simulink model "plantaCPC_2025_PLC"  (R2025b)
settings: Solver=ode45  StartTime=0.0  StopTime=300  MaxStep=0.01  RelTol=1e-5  EnableMultiTasking=on
values from neighbouring files (symbols this model uses):
  A = 0.159    [Fuzzy_no_anfis_sim.m]    (also in build_FLC_L4_anfis.m = zeros(size(Xtr,1), nOut); build_FLC_lower_single.m; build_FLC_upper_single.m; fuzzym.m)
  a1 = 6.1360e-04    (= 0.0006136)    [Fuzzy_no_anfis_sim.m]    (also in build_FLC_lower_single.m; fuzzym.m)
  a2 = 5.4678e-04    (= 0.00054678)    [Fuzzy_no_anfis_sim.m]    (also in build_FLC_lower_single.m; fuzzym.m)
  a3 = 3.5752e-04    (= 0.00035752)    [Fuzzy_no_anfis_sim.m]    (also in build_FLC_lower_single.m; fuzzym.m)
  a4 = 4.1820e-04    (= 0.0004182)    [Fuzzy_no_anfis_sim.m]    (also in build_FLC_L4_anfis.m; build_FLC_L4_single.m; build_FLC_lower_single.m; fuzzym.m)
  dumax = 1    [Fuzzy_no_anfis_sim.m]
  gamma1 = 0.455    [Fuzzy_no_anfis_sim.m]    (also in build_FLC_L4_anfis.m; build_FLC_L4_single.m; build_FLC_lower_single.m; fuzzym.m)
  gamma2 = 0.4195    [Fuzzy_no_anfis_sim.m]    (also in build_FLC_lower_single.m; fuzzym.m)
  k1 = q_max    (= 0.0017)    [Fuzzy_no_anfis_sim.m]    (also in build_FLC_L4_anfis.m; build_FLC_L4_single.m; fuzzym.m)
  k2 = q_max    (= 0.0017)    [Fuzzy_no_anfis_sim.m]    (also in fuzzym.m)
  Ts = 0.1    [Fuzzy_no_anfis_sim.m]    (also in build_FLC_L4_single.m; build_FLC_lower_single.m; build_FLC_upper_single.m; deadbeat_flc_pump2.m = 1)
undefined symbols (not defined in the file or in its folder): dspblkCoreblockFVToolHelper, gcbh
libraries: simulink x30, fuzblock x4
settings Model: PacingRate=3  Creator=Administrator  LastModifiedBy=wepi
settings DataIOCC: LimitDataPoints=on  SaveFormat=Array  ReturnWorkspaceOutputs=off
settings OptimizationCC: LifeSpan=inf
settings DebuggingCC: UnderspecifiedInitializationDetection=Classic  MergeDetectMultiDrivingBlocksExec=none  SolverPrmCheckMsg=warning  UnconnectedInputMsg=warning  UnconnectedOutputMsg=warning  UnconnectedLineMsg=warning  StateNameClashWarn=warning  SFUnexpectedBacktrackingDiag=warning  SFNoUnconditionalDefaultTransitionDiag=warning  SFExecutionAtInitializationDiag=none  ArithmeticOperatorsInVariantConditions=warning
settings HardwareCC: ProdBitPerPointer=32.0  ProdBitPerSizeT=32.0  ProdBitPerPtrDiffT=32.0  ProdLargestAtomicFloat=None  ProdIntDivRoundTo=Undefined  ProdEndianess=Unspecified  ProdWordSize=32.0  ProdHWDeviceType=32-bit Generic
settings ModelReferenceCC: PropagateSignalLabelsOutOfModel=off
settings SFSimCC: SimUseLocalCustomCode=off  CustomCodeUndefinedFunction=UseInterfaceOnly
settings RTWCC: RTWUseLocalCustomCode=off  GPUComputeCapability=3.5
settings CodeAppCC: StateflowObjectComments=on
settings GRTTargetCC: TargetLangStandard=C89/C90 (ANSI)
settings ConfigComp: CovMetricSettings=dw  CovSaveCumulativeToWorkspaceVar=on  CovSaveSingleToWorkspaceVar=on  CovExternalEMLEnable=off

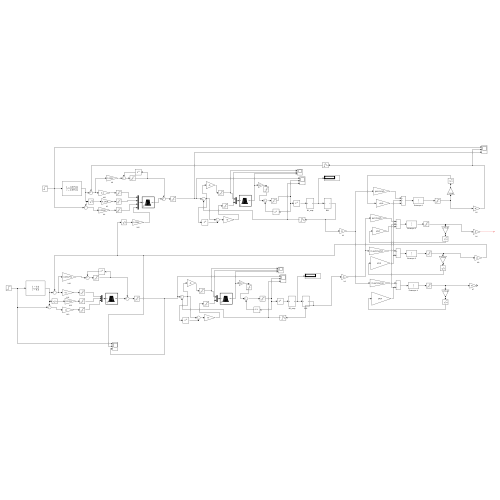
[thumbnail: Simulink's stored preview of the top-level diagram]
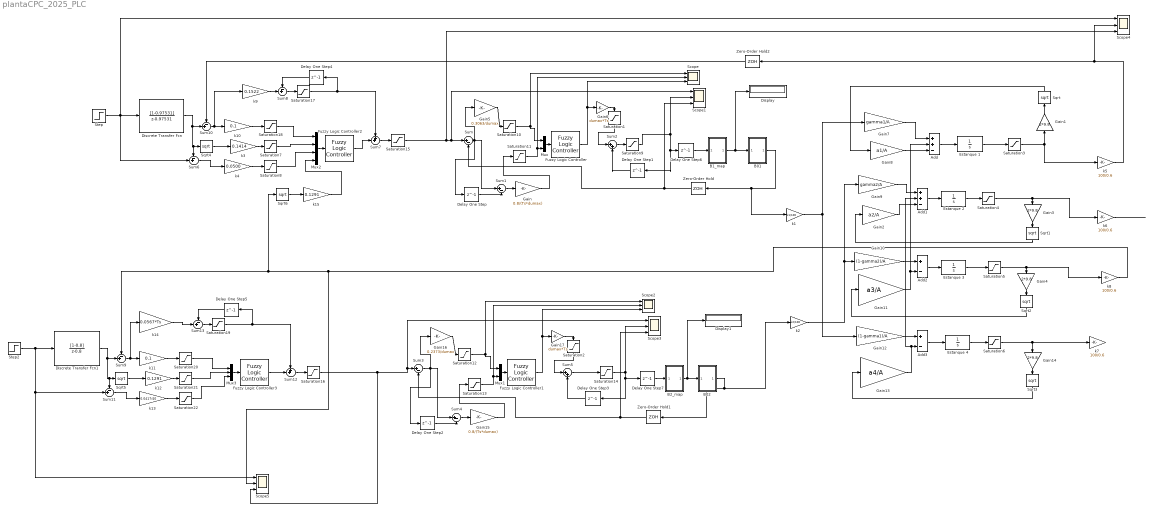
== system plantaCPC_2025_PLC ==
  Add : Sum  Inputs=++-
  Add1 : Sum  Inputs=++-
  Add2 : Sum  Inputs=+-
  Add3 : Sum  Inputs=+-
  B01 : Subsystem
  B02 : Subsystem
  B1_map : Subsystem
  B2_map : Subsystem
  Delay One Step{,2,6..7} (4 alike) : Delay  DelayLength=1  SampleTime=0.1
  Delay One Step1 : Delay  DelayLength=1  InitialCondition=0  SampleTime=0.1
  Delay One Step3 : Delay  DelayLength=1  InitialCondition=40  SampleTime=0.1
  Delay One Step4 : Delay  DelayLength=1  InitialCondition=0  SampleTime=0.1
  Delay One Step5 : Delay  DelayLength=1  InitialCondition=0  SampleTime=0.1
  Discrete Transfer Fcn : DiscreteTransferFcn  LoadFcn=dspblkCoreblockFVToolHelper(gcbh,'load');  Numerator=[1-0.97531]  Denominator=[1 -0.97531]
      settings: CopyFcn=dspblkCoreblockFVToolHelper(gcbh,'copy');  DeleteFcn=dspblkCoreblockFVToolHelper(gcbh,'close');  ModelCloseFcn=dspblkCoreblockFVToolHelper(gcbh,'close');  PreSaveFcn=dspblkCoreblockFVToolHelper(gcbh,'presave');  PostSaveFcn=dspblkCoreblockFVToolHelper(gcbh,'postsave');  CloseFcn=dspblkCoreblockFVToolHelper(gcbh,'close');
  Discrete Transfer Fcn1 : DiscreteTransferFcn  LoadFcn=dspblkCoreblockFVToolHelper(gcbh,'load');  Numerator=[1-0.8]  Denominator=[1 -0.8]
      settings: CopyFcn=dspblkCoreblockFVToolHelper(gcbh,'copy');  DeleteFcn=dspblkCoreblockFVToolHelper(gcbh,'close');  ModelCloseFcn=dspblkCoreblockFVToolHelper(gcbh,'close');  PreSaveFcn=dspblkCoreblockFVToolHelper(gcbh,'presave');  PostSaveFcn=dspblkCoreblockFVToolHelper(gcbh,'postsave');  CloseFcn=dspblkCoreblockFVToolHelper(gcbh,'close');
  Display : Display
  Display1 : Display
  Estanque 1 : TransferFcn  Denominator=[1 0]
  "Estanque 2 " : TransferFcn  Denominator=[1 0]
  Estanque 3 : TransferFcn  Denominator=[1 0]
  Estanque 4 : TransferFcn  Denominator=[1 0]
  Fuzzy Logic Controller : fuzblock/Fuzzy Logic  Controller  FIS=FLC_F1  OutputSampleNumber=101  DataType=double  UseLookupTable=off  NumBreakpoints=10  FuzzifiedInputs=off  RuleFiringStrengths=off  RuleOutputs=off  AggregatedOutputs=off  SimulateUsing=Interpreted execution  OutOfRangeInputValueMessage=warning  NoRuleFiredMessage=warning  EmptyOutputFuzzySetMessage=warning
  Fuzzy Logic Controller1 : fuzblock/Fuzzy Logic  Controller  FIS=FLC_F2  OutputSampleNumber=101  DataType=double  UseLookupTable=off  NumBreakpoints=10  FuzzifiedInputs=off  RuleFiringStrengths=off  RuleOutputs=off  AggregatedOutputs=off  SimulateUsing=Interpreted execution  OutOfRangeInputValueMessage=warning  NoRuleFiredMessage=warning  EmptyOutputFuzzySetMessage=warning
  Fuzzy Logic Controller2 : fuzblock/Fuzzy Logic  Controller  FIS=FLC_L1  OutputSampleNumber=101  DataType=double  UseLookupTable=off  NumBreakpoints=10  FuzzifiedInputs=off  RuleFiringStrengths=off  RuleOutputs=off  AggregatedOutputs=off  SimulateUsing=Interpreted execution  OutOfRangeInputValueMessage=warning  NoRuleFiredMessage=warning  EmptyOutputFuzzySetMessage=warning
  Fuzzy Logic Controller3 : fuzblock/Fuzzy Logic  Controller  FIS=FLC_L3  OutputSampleNumber=101  DataType=double  UseLookupTable=off  NumBreakpoints=10  FuzzifiedInputs=off  RuleFiringStrengths=off  RuleOutputs=off  AggregatedOutputs=off  SimulateUsing=Interpreted execution  OutOfRangeInputValueMessage=warning  NoRuleFiredMessage=warning  EmptyOutputFuzzySetMessage=warning
  Gain : Gain  Gain=0.8/(Ts*dumax)
  Gain{1,3..4,14} (4 alike) : Gain  Gain=2*9.8
  Gain10 : Gain  Gain=(1-gamma2)/A
  Gain11 : Gain  Gain=a3/A
  Gain12 : Gain  Gain=(1-gamma1)/A
  Gain13 : Gain  Gain=a4/A
  Gain15 : Gain  Gain=0.8/(Ts*dumax)
  Gain16 : Gain  Gain=0.2373/dumax
  Gain17 : Gain  Gain=dumax*Ts
  Gain2 : Gain  Gain=a2/A
  Gain5 : Gain  Gain=0.3063/dumax
  Gain6 : Gain  Gain=dumax*Ts
  Gain7 : Gain  Gain=gamma1/A
  Gain8 : Gain  Gain=a1/A
  Gain9 : Gain  Gain=gamma2/A
  Mux : Mux  Inputs=2
  Mux1 : Mux  Inputs=2
  Mux2 : Mux
  Mux3 : Mux  Inputs=3
  Saturation1 : Saturate  UpperLimit=dumax*Ts  LowerLimit=-dumax*Ts
  Saturation{8,10..13,18,20,22} (8 alike) : Saturate  UpperLimit=1  LowerLimit=-1
  Saturation{9,14..16} (4 alike) : Saturate  UpperLimit=100  LowerLimit=0
  Saturation17 : Saturate  UpperLimit=30  LowerLimit=-30
  Saturation19 : Saturate  UpperLimit=30  LowerLimit=-30
  Saturation2 : Saturate  UpperLimit=dumax*Ts  LowerLimit=-dumax*Ts
  Saturation21 : Saturate  UpperLimit=1  LowerLimit=0
  Saturation{3..6} (4 alike) : Saturate  UpperLimit=0.8  LowerLimit=0
  Saturation7 : Saturate  UpperLimit=1  LowerLimit=0
  Scope{,1..5} (6 alike) : Scope  NumInputPorts=3
      Scope settings: ActiveDisplayYMinimum=103.80137956396959  ActiveDisplayYMaximum=139.96234120398589
      Scope1 settings: ActiveDisplayYMinimum=-68.909700061778238  ActiveDisplayYMaximum=113.12239490018993
      Scope2 settings: ActiveDisplayYMinimum=103.80137956396959  ActiveDisplayYMaximum=139.96234120398589  DataLoggingVariableName=ScopeData2
      Scope3 settings: ActiveDisplayYMinimum=-52.0727443173749  ActiveDisplayYMaximum=103.1546988563742  DataLoggingVariableName=ScopeData3
      Scope4 settings: ActiveDisplayYMinimum=-77.521735134950461  ActiveDisplayYMaximum=137.02283230652165  DataLoggingVariableName=ScopeData4
      Scope5 settings: ActiveDisplayYMinimum=-10.950989781729737  ActiveDisplayYMaximum=98.55890803556764  DataLoggingVariableName=ScopeData5
  Sqrt{,1..6} (7 alike) : Sqrt
  Step : Step  Time=200  Before=10  After=20  SampleTime=0
  Step2 : Step  Time=90  Before=10  After=20  SampleTime=0
  Sum{,1,3..4} (4 alike) : Sum  Inputs=|+-
  Sum{6,8..11,13} (6 alike) : Sum  Inputs=-+|
  Sum12 : Sum  Inputs=++|
  Sum2 : Sum  Inputs=|++
  Sum5 : Sum  Inputs=|++
  Sum7 : Sum  Inputs=++|
  Zero-Order Hold : ZeroOrderHold  SampleTime=Ts
  Zero-Order Hold1 : ZeroOrderHold  SampleTime=Ts
  Zero-Order Hold2 : ZeroOrderHold  SampleTime=Ts
  k1 : Gain  Gain=k1/100
  k10 : Gain  Gain=0.1
  k11 : Gain  Gain=0.1
  k12 : Gain  Gain=0.1291
  k13 : Gain  Gain=0.0417/40
  k14 : Gain  Gain=0.0567*Ts
  k15 : Gain  Gain=0.1291
  k2 : Gain  Gain=k2/100
  k3 : Gain  Gain=0.1414
  k4 : Gain  Gain=0.0500
  k{5..8} (4 alike) : Gain  Gain=100/0.6
  k9 : Gain  Gain=0.1522
  wires:
  Saturation3/1 -> k5/1, Gain1/1
  Saturation4/1 -> k6/1, Gain3/1
  Saturation5/1 -> k8/1, Gain4/1
  Estanque 1/1 -> Saturation3/1
  "Estanque 2 "/1 -> Saturation4/1
  Estanque 4/1 -> Saturation6/1
  Fuzzy Logic Controller/1 -> Gain6/1, Scope/3
  Gain7/1 -> Add/1
  k1/1 -> Gain12/1, Gain7/1
  Gain8/1 -> Add/3
  Add/1 -> Estanque 1/1
  Add1/1 -> "Estanque 2 "/1
  Add2/1 -> Estanque 3/1
  Add3/1 -> Estanque 4/1
  Gain9/1 -> Add1/1
  k2/1 -> Gain9/1, Gain10/1
  Gain2/1 -> Add1/3
  Gain10/1 -> Add2/1
  Gain11/1 -> Add/2, Add2/2
  Gain12/1 -> Add3/1
  Gain13/1 -> Add1/2, Add3/2
  Estanque 3/1 -> Saturation5/1
  Gain1/1 -> Sqrt/1
  Sqrt/1 -> Gain8/1
  Gain3/1 -> Sqrt1/1
  Sqrt1/1 -> Gain2/1
  Gain4/1 -> Sqrt2/1
  Gain14/1 -> Sqrt3/1
  Saturation6/1 -> Gain14/1, k7/1
  Sqrt3/1 -> Gain13/1
  Sqrt2/1 -> Gain11/1
  Sum2/1 -> Saturation9/1
  k6/1 -> ?
  Sum/1 -> Delay One Step/1, Gain5/1, Sum1/1
  Mux/1 -> Fuzzy Logic Controller/1
  Delay One Step/1 -> Sum1/2
  Saturation11/1 -> Scope/2, Mux/2
  Saturation10/1 -> Scope/1, Mux/1
  Saturation9/1 -> Delay One Step1/1, Delay One Step6/1, Scope1/2
  B01/1(Out1) -> k1/1, Zero-Order Hold/1
  Gain6/1 -> Saturation1/1
  Saturation1/1 -> Sum2/1
  Delay One Step1/1 -> Sum2/2
  Gain5/1 -> Saturation10/1
  Sum1/1 -> Gain/1
  Gain/1 -> Saturation11/1
  B1_map/1(Out1) -> Display/1, B01/1(In1)
  Zero-Order Hold/1 -> Sum/2, Scope1/3
  Mux1/1 -> Fuzzy Logic Controller1/1
  Sum5/1 -> Saturation14/1
  Delay One Step3/1 -> Sum5/2
  Sum4/1 -> Gain15/1
  B2_map/1(Out1) -> Display1/1, B02/1(In1)
  Gain16/1 -> Saturation12/1
  B02/1(Out1) -> Zero-Order Hold1/1, k2/1
  Fuzzy Logic Controller1/1 -> Gain17/1, Scope2/3
  Zero-Order Hold1/1 -> Sum3/2, Scope3/3
  Sum3/1 -> Delay One Step2/1, Gain16/1, Sum4/1
  Saturation13/1 -> Scope2/2, Mux1/2
  Delay One Step2/1 -> Sum4/2
  Gain15/1 -> Saturation13/1
  Saturation16/1 -> Scope5/3, Scope3/1, Sum3/1
  Gain17/1 -> Saturation2/1
  Saturation2/1 -> Sum5/1
  Saturation12/1 -> Scope2/1, Mux1/1
  Saturation14/1 -> Delay One Step7/1, Delay One Step3/1, Scope3/2
  Mux2/1 -> Fuzzy Logic Controller2/1
  Fuzzy Logic Controller2/1 -> Sum7/2
  Saturation15/1 -> Scope4/3, Scope1/1, Sum/1
  Delay One Step6/1 -> B1_map/1(In1)
  Step/1 -> Sum6/2, Scope4/1, Discrete Transfer Fcn/1
  Discrete Transfer Fcn/1 -> Sum6/1, Sqrt4/1, Sum10/2
  Sum10/1 -> k9/1, k10/1
  k10/1 -> Saturation18/1
  Saturation18/1 -> Mux2/1
  Zero-Order Hold2/1 -> Sum10/1
  Sum7/1 -> Saturation15/1
  k3/1 -> Saturation7/1
  Saturation7/1 -> Mux2/2
  Sum6/1 -> k4/1
  k4/1 -> Saturation8/1
  Saturation8/1 -> Mux2/3
  k9/1 -> Sum8/2
  Sum8/1 -> Saturation17/1
  Saturation17/1 -> Delay One Step4/1, Sum7/1
  Delay One Step4/1 -> Sum8/1
  Sqrt4/1 -> k3/1
  Sum12/1 -> Saturation16/1
  k13/1 -> Saturation22/1
  Mux3/1 -> Fuzzy Logic Controller3/1
  k12/1 -> Saturation21/1
  Fuzzy Logic Controller3/1 -> Sum12/2
  Saturation21/1 -> Mux3/2
  Sum13/1 -> Saturation19/1
  Step2/1 -> Scope5/1, Sum11/2, Discrete Transfer Fcn1/1
  Saturation22/1 -> Mux3/3
  k14/1 -> Sum13/2
  k11/1 -> Saturation20/1
  Discrete Transfer Fcn1/1 -> Sum11/1, Sqrt5/1, Sum9/2
  Sum9/1 -> k14/1, k11/1
  Sqrt5/1 -> k12/1
  Saturation19/1 -> Delay One Step5/1, Sum12/1
  Saturation20/1 -> Mux3/1
  Delay One Step5/1 -> Sum13/1
  Sum11/1 -> k13/1
  k8/1 -> Scope5/2, Sqrt6/1, Sum9/1
  Delay One Step7/1 -> B2_map/1(In1)
  Sqrt6/1 -> k15/1
  k15/1 -> Mux2/4
  k5/1 -> Scope4/2, Zero-Order Hold2/1

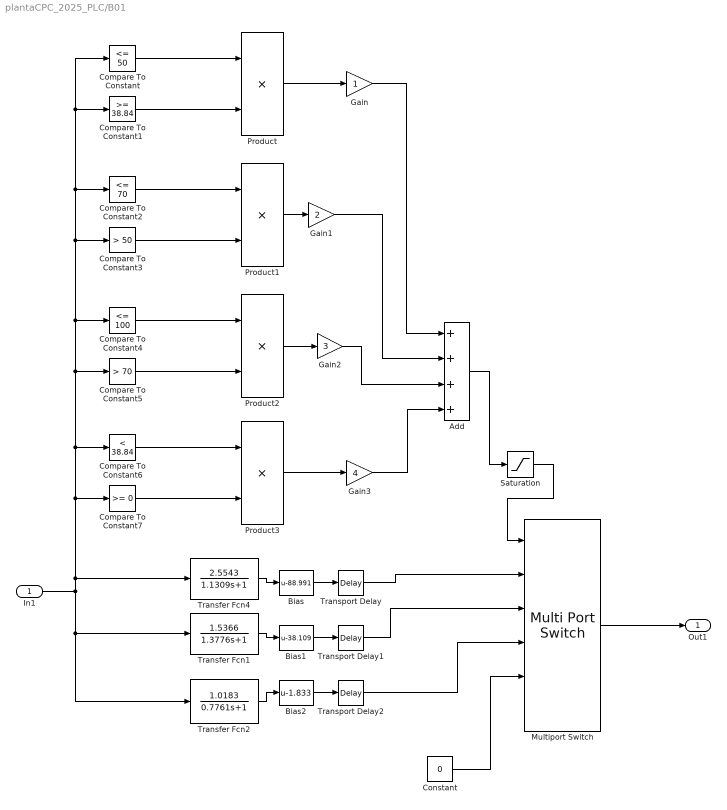
== system plantaCPC_2025_PLC/B01 ==
  In1 : Inport
  Add : Sum  Inputs=++++
  Bias : Bias  Bias=-88.991  SaturateOnIntegerOverflow=off
  Bias1 : Bias  Bias=-38.109  SaturateOnIntegerOverflow=off
  Bias2 : Bias  Bias=-1.833  SaturateOnIntegerOverflow=off
  Compare To Constant : simulink/Logic and Bit Operations/Compare To Constant  relop=<=  const=50  OutDataTypeStr=boolean
  Compare To Constant1 : simulink/Logic and Bit Operations/Compare To Constant  relop=>=  const=38.84  OutDataTypeStr=boolean
  Compare To Constant2 : simulink/Logic and Bit Operations/Compare To Constant  relop=<=  const=70  OutDataTypeStr=boolean
  Compare To Constant3 : simulink/Logic and Bit Operations/Compare To Constant  relop=>  const=50  OutDataTypeStr=boolean
  Compare To Constant4 : simulink/Logic and Bit Operations/Compare To Constant  relop=<=  const=100  OutDataTypeStr=boolean
  Compare To Constant5 : simulink/Logic and Bit Operations/Compare To Constant  relop=>  const=70  OutDataTypeStr=boolean
  Compare To Constant6 : simulink/Logic and Bit Operations/Compare To Constant  relop=<  const=38.84  OutDataTypeStr=boolean
  Compare To Constant7 : simulink/Logic and Bit Operations/Compare To Constant  relop=>=  const=0  OutDataTypeStr=boolean
  Constant : Constant  Value=0
  Gain : Gain
  Gain1 : Gain  Gain=2
  Gain2 : Gain  Gain=3
  Gain3 : Gain  Gain=4
  Multiport Switch : MultiPortSwitch  Inputs=5  SaturateOnIntegerOverflow=off  InputSameDT=off
  Product{,1..3} (4 alike) : Product
  Saturation : Saturate  UpperLimit=5  LowerLimit=1
  Transfer Fcn1 : TransferFcn  Numerator=[1.5366]  Denominator=[1.3776 1]
  Transfer Fcn2 : TransferFcn  Numerator=[1.0183]  Denominator=[0.7761 1]
  Transfer Fcn4 : TransferFcn  Numerator=[2.5543]  Denominator=[1.1309 1]
  Transport Delay : TransportDelay  DelayTime=0.6
  Transport Delay1 : TransportDelay  DelayTime=0.5
  Transport Delay2 : TransportDelay  DelayTime=0.5
  Out1 : Outport
  wires:
  Multiport Switch/1 -> Out1/1
  Product/1 -> Gain/1
  Gain/1 -> Add/1
  Product1/1 -> Gain1/1
  Gain1/1 -> Add/2
  Gain2/1 -> Add/3
  Product2/1 -> Gain2/1
  Add/1 -> Saturation/1
  Compare To Constant/1 -> Product/1
  Transfer Fcn4/1 -> Bias/1
  Transfer Fcn1/1 -> Bias1/1
  Transfer Fcn2/1 -> Bias2/1
  Compare To Constant1/1 -> Product/2
  Compare To Constant2/1 -> Product1/1
  Compare To Constant3/1 -> Product1/2
  Compare To Constant4/1 -> Product2/1
  Compare To Constant5/1 -> Product2/2
  Transport Delay1/1 -> Multiport Switch/3
  Transport Delay2/1 -> Multiport Switch/4
  Bias/1 -> Transport Delay/1
  Bias1/1 -> Transport Delay1/1
  Bias2/1 -> Transport Delay2/1
  Product3/1 -> Gain3/1
  Compare To Constant6/1 -> Product3/1
  Compare To Constant7/1 -> Product3/2
  In1/1 -> Compare To Constant7/1, Compare To Constant6/1, Compare To Constant4/1, Compare To Constant2/1, Compare To Constant1/1, Compare To Constant/1, Compare To Constant3/1, Compare To Constant5/1, Transfer Fcn4/1, Transfer Fcn2/1, Transfer Fcn1/1
  Gain3/1 -> Add/4
  Constant/1 -> Multiport Switch/5
  Transport Delay/1 -> Multiport Switch/2
  Saturation/1 -> Multiport Switch/1

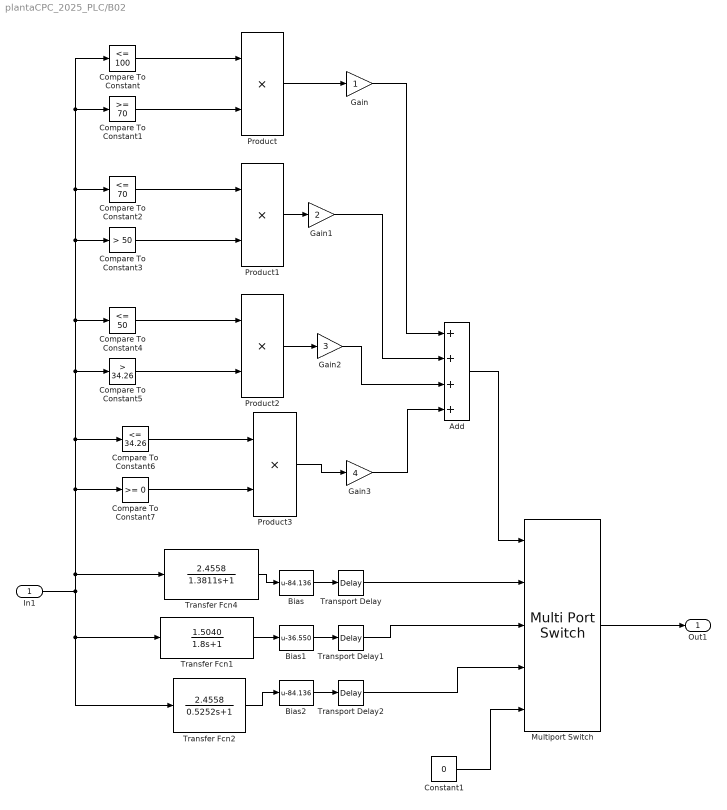
== system plantaCPC_2025_PLC/B02 ==
  In1 : Inport
  Add : Sum  Inputs=++++
  Bias : Bias  Bias=-84.136  SaturateOnIntegerOverflow=off
  Bias1 : Bias  Bias=-36.550  SaturateOnIntegerOverflow=off
  Bias2 : Bias  Bias=-84.136  SaturateOnIntegerOverflow=off
  Compare To Constant : simulink/Logic and Bit Operations/Compare To Constant  relop=<=  const=100  OutDataTypeStr=boolean
  Compare To Constant1 : simulink/Logic and Bit Operations/Compare To Constant  relop=>=  const=70  OutDataTypeStr=boolean
  Compare To Constant2 : simulink/Logic and Bit Operations/Compare To Constant  relop=<=  const=70  OutDataTypeStr=boolean
  Compare To Constant3 : simulink/Logic and Bit Operations/Compare To Constant  relop=>  const=50  OutDataTypeStr=boolean
  Compare To Constant4 : simulink/Logic and Bit Operations/Compare To Constant  relop=<=  const=50  OutDataTypeStr=boolean
  Compare To Constant5 : simulink/Logic and Bit Operations/Compare To Constant  relop=>  const=34.26  OutDataTypeStr=boolean
  Compare To Constant6 : simulink/Logic and Bit Operations/Compare To Constant  relop=<=  const=34.26  OutDataTypeStr=boolean
  Compare To Constant7 : simulink/Logic and Bit Operations/Compare To Constant  relop=>=  const=0  OutDataTypeStr=boolean
  Constant1 : Constant  Value=0
  Gain : Gain
  Gain1 : Gain  Gain=2
  Gain2 : Gain  Gain=3
  Gain3 : Gain  Gain=4
  Multiport Switch : MultiPortSwitch  Inputs=4  SaturateOnIntegerOverflow=off  InputSameDT=off
  Product{,1..3} (4 alike) : Product
  Transfer Fcn1 : TransferFcn  Numerator=[1.5040]  Denominator=[1.8 1]
  Transfer Fcn2 : TransferFcn  Numerator=[2.4558]  Denominator=[0.5252 1]
  Transfer Fcn4 : TransferFcn  Numerator=[2.4558]  Denominator=[1.3811 1]
  Transport Delay : TransportDelay  DelayTime=0.5
  Transport Delay1 : TransportDelay  DelayTime=0.5
  Transport Delay2 : TransportDelay  DelayTime=0.8
  Out1 : Outport
  wires:
  Multiport Switch/1 -> Out1/1
  Product/1 -> Gain/1
  Gain/1 -> Add/1
  Product1/1 -> Gain1/1
  Gain1/1 -> Add/2
  Gain2/1 -> Add/3
  Product2/1 -> Gain2/1
  Add/1 -> Multiport Switch/1
  Compare To Constant/1 -> Product/1
  Transfer Fcn4/1 -> Bias/1
  Transfer Fcn1/1 -> Bias1/1
  Transfer Fcn2/1 -> Bias2/1
  Compare To Constant1/1 -> Product/2
  Compare To Constant2/1 -> Product1/1
  Compare To Constant3/1 -> Product1/2
  Compare To Constant4/1 -> Product2/1
  Compare To Constant5/1 -> Product2/2
  Transport Delay/1 -> Multiport Switch/2
  Transport Delay1/1 -> Multiport Switch/3
  Transport Delay2/1 -> Multiport Switch/4
  Bias/1 -> Transport Delay/1
  Bias1/1 -> Transport Delay1/1
  Bias2/1 -> Transport Delay2/1
  Gain3/1 -> Add/4
  Constant1/1 -> Multiport Switch/5
  Compare To Constant7/1 -> Product3/2
  Compare To Constant6/1 -> Product3/1
  In1/1 -> Compare To Constant7/1, Compare To Constant6/1, Compare To Constant4/1, Compare To Constant2/1, Compare To Constant1/1, Compare To Constant/1, Compare To Constant3/1, Compare To Constant5/1, Transfer Fcn4/1, Transfer Fcn2/1, Transfer Fcn1/1
  Product3/1 -> Gain3/1

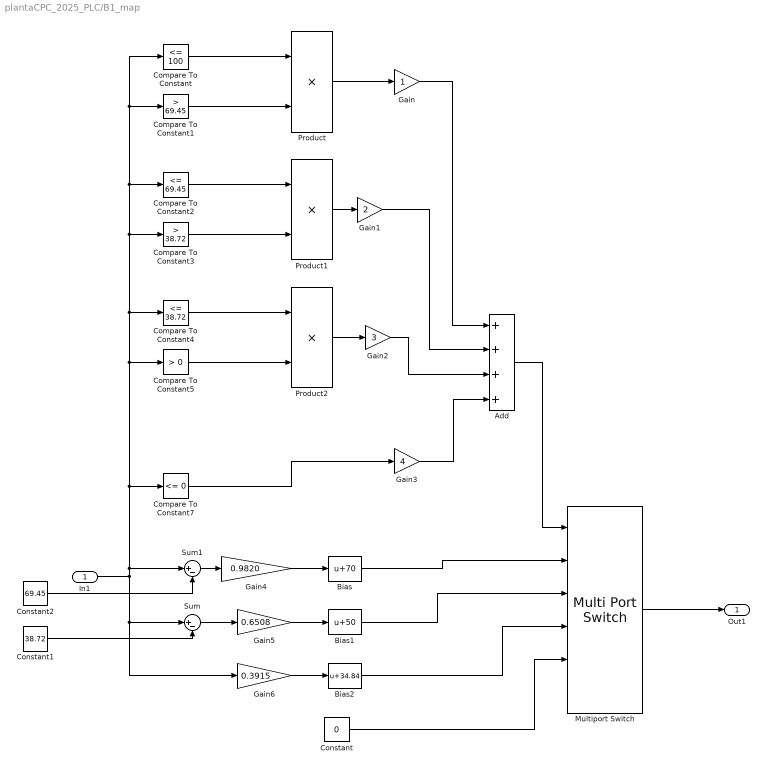
== system plantaCPC_2025_PLC/B1_map ==
  In1 : Inport
  Add : Sum  Inputs=++++
  Bias : Bias  Bias=70  SaturateOnIntegerOverflow=off
  Bias1 : Bias  Bias=50  SaturateOnIntegerOverflow=off
  Bias2 : Bias  Bias=34.84  SaturateOnIntegerOverflow=off
  Compare To Constant : simulink/Logic and Bit Operations/Compare To Constant  relop=<=  const=100  OutDataTypeStr=boolean
  Compare To Constant1 : simulink/Logic and Bit Operations/Compare To Constant  relop=>  const=69.45  OutDataTypeStr=boolean
  Compare To Constant2 : simulink/Logic and Bit Operations/Compare To Constant  relop=<=  const=69.45  OutDataTypeStr=boolean
  Compare To Constant3 : simulink/Logic and Bit Operations/Compare To Constant  relop=>  const=38.72  OutDataTypeStr=boolean
  Compare To Constant4 : simulink/Logic and Bit Operations/Compare To Constant  relop=<=  const=38.72  OutDataTypeStr=boolean
  Compare To Constant5 : simulink/Logic and Bit Operations/Compare To Constant  relop=>  const=0  OutDataTypeStr=boolean
  Compare To Constant7 : simulink/Logic and Bit Operations/Compare To Constant  relop=<=  const=0  OutDataTypeStr=boolean
  Constant : Constant  Value=0
  Constant1 : Constant  Value=38.72
  Constant2 : Constant  Value=69.45
  Gain : Gain
  Gain1 : Gain  Gain=2
  Gain2 : Gain  Gain=3
  Gain3 : Gain  Gain=4
  Gain4 : Gain  Gain=0.9820
  Gain5 : Gain  Gain=0.6508
  Gain6 : Gain  Gain=0.3915
  Multiport Switch : MultiPortSwitch  Inputs=5  SaturateOnIntegerOverflow=off  InputSameDT=off
  Product : Product
  Product1 : Product
  Product2 : Product
  Sum : Sum  Inputs=|+-
  Sum1 : Sum  Inputs=|+-
  Out1 : Outport
  wires:
  Bias/1 -> Multiport Switch/2
  Constant/1 -> Multiport Switch/5
  Gain3/1 -> Add/4
  Compare To Constant7/1 -> Gain3/1
  Bias2/1 -> Multiport Switch/4
  Bias1/1 -> Multiport Switch/3
  Compare To Constant5/1 -> Product2/2
  Compare To Constant4/1 -> Product2/1
  Compare To Constant3/1 -> Product1/2
  Compare To Constant2/1 -> Product1/1
  Compare To Constant1/1 -> Product/2
  In1/1 -> Sum/1, Gain6/1, Sum1/1, Compare To Constant5/1, Compare To Constant3/1, Compare To Constant/1, Compare To Constant1/1, Compare To Constant2/1, Compare To Constant4/1, Compare To Constant7/1
  Gain5/1 -> Bias1/1
  Gain4/1 -> Bias/1
  Compare To Constant/1 -> Product/1
  Add/1 -> Multiport Switch/1
  Product2/1 -> Gain2/1
  Gain2/1 -> Add/3
  Gain1/1 -> Add/2
  Product1/1 -> Gain1/1
  Gain/1 -> Add/1
  Product/1 -> Gain/1
  Multiport Switch/1 -> Out1/1
  Gain6/1 -> Bias2/1
  Sum/1 -> Gain5/1
  Sum1/1 -> Gain4/1
  Constant1/1 -> Sum/2
  Constant2/1 -> Sum1/2

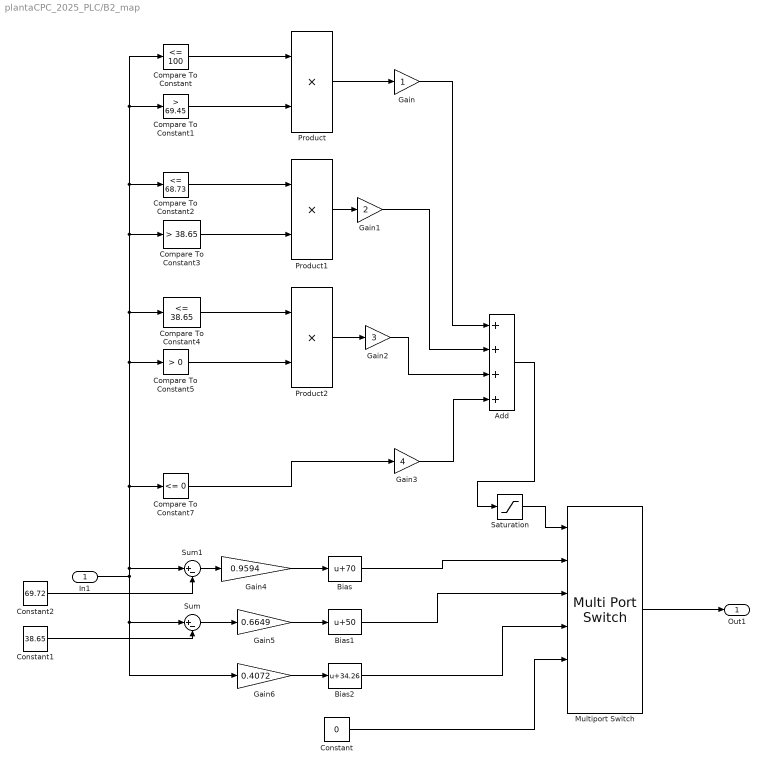
== system plantaCPC_2025_PLC/B2_map ==
  In1 : Inport
  Add : Sum  Inputs=++++
  Bias : Bias  Bias=70  SaturateOnIntegerOverflow=off
  Bias1 : Bias  Bias=50  SaturateOnIntegerOverflow=off
  Bias2 : Bias  Bias=34.26  SaturateOnIntegerOverflow=off
  Compare To Constant : simulink/Logic and Bit Operations/Compare To Constant  relop=<=  const=100  OutDataTypeStr=boolean
  Compare To Constant1 : simulink/Logic and Bit Operations/Compare To Constant  relop=>  const=69.45  OutDataTypeStr=boolean
  Compare To Constant2 : simulink/Logic and Bit Operations/Compare To Constant  relop=<=  const=68.73  OutDataTypeStr=boolean
  Compare To Constant3 : simulink/Logic and Bit Operations/Compare To Constant  relop=>  const=38.65  OutDataTypeStr=boolean
  Compare To Constant4 : simulink/Logic and Bit Operations/Compare To Constant  relop=<=  const=38.65  OutDataTypeStr=boolean
  Compare To Constant5 : simulink/Logic and Bit Operations/Compare To Constant  relop=>  const=0  OutDataTypeStr=boolean
  Compare To Constant7 : simulink/Logic and Bit Operations/Compare To Constant  relop=<=  const=0  OutDataTypeStr=boolean
  Constant : Constant  Value=0
  Constant1 : Constant  Value=38.65
  Constant2 : Constant  Value=69.72
  Gain : Gain
  Gain1 : Gain  Gain=2
  Gain2 : Gain  Gain=3
  Gain3 : Gain  Gain=4
  Gain4 : Gain  Gain=0.9594
  Gain5 : Gain  Gain=0.6649
  Gain6 : Gain  Gain=0.4072
  Multiport Switch : MultiPortSwitch  Inputs=5  SaturateOnIntegerOverflow=off  InputSameDT=off
  Product : Product
  Product1 : Product
  Product2 : Product
  Saturation : Saturate  UpperLimit=5  LowerLimit=1
  Sum : Sum  Inputs=|+-
  Sum1 : Sum  Inputs=|+-
  Out1 : Outport
  wires:
  Constant2/1 -> Sum1/2
  Constant1/1 -> Sum/2
  Sum1/1 -> Gain4/1
  Sum/1 -> Gain5/1
  Gain6/1 -> Bias2/1
  Multiport Switch/1 -> Out1/1
  Product/1 -> Gain/1
  Gain/1 -> Add/1
  Product1/1 -> Gain1/1
  Gain1/1 -> Add/2
  Gain2/1 -> Add/3
  Product2/1 -> Gain2/1
  Add/1 -> Saturation/1
  Compare To Constant/1 -> Product/1
  Gain4/1 -> Bias/1
  Gain5/1 -> Bias1/1
  In1/1 -> Compare To Constant7/1, Compare To Constant4/1, Compare To Constant2/1, Compare To Constant1/1, Compare To Constant/1, Compare To Constant3/1, Compare To Constant5/1, Sum1/1, Gain6/1, Sum/1
  Compare To Constant1/1 -> Product/2
  Compare To Constant2/1 -> Product1/1
  Compare To Constant3/1 -> Product1/2
  Compare To Constant4/1 -> Product2/1
  Compare To Constant5/1 -> Product2/2
  Bias1/1 -> Multiport Switch/3
  Bias2/1 -> Multiport Switch/4
  Compare To Constant7/1 -> Gain3/1
  Gain3/1 -> Add/4
  Constant/1 -> Multiport Switch/5
  Bias/1 -> Multiport Switch/2
  Saturation/1 -> Multiport Switch/1
